simulink model "fourier"  (Simulink 6.3)
settings: Solver=ode45  StartTime=0.0  StopTime=10.0  RelTol=1e-3
settings Model: LastModifiedBy=33242

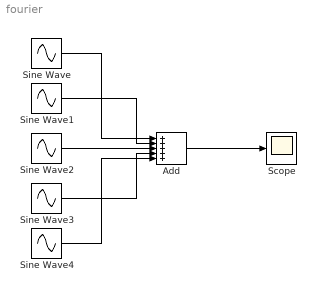
== system fourier ==
  Add : Sum  Inputs=+++++  OutScaling=2^-10
  Scope : Scope
  Sine Wave : Sin  Frequency=2*pi  SampleTime=0
  Sine Wave1 : Sin  Amplitude=1/3  Frequency=3*2*pi  SampleTime=0
  Sine Wave2 : Sin  Amplitude=1/5  Frequency=5*2*pi  SampleTime=0
  Sine Wave3 : Sin  Amplitude=1/7  Frequency=7*2*pi  SampleTime=0
  Sine Wave4 : Sin  Amplitude=1/9  Frequency=9*2*pi  SampleTime=0
  wires:
  Sine Wave2/1 -> Add/3
  Sine Wave/1 -> Add/1
  Sine Wave4/1 -> Add/5
  Sine Wave3/1 -> Add/4
  Sine Wave1/1 -> Add/2
  Add/1 -> Scope/1
